simulink model "TemperatureControl"  (R2024b)
settings: Solver=FixedStepAuto  StartTime=0.0  StopTime=inf  FixedStep=0.1  RelTol=1e-3  EnableMultiTasking=on
libraries: arduinolib x6
settings Model: ExtModeTrigDuration=2  Creator=arkad  LastModifiedBy=arkad
settings SolverCC: AutoInsertRateTranBlk=on
settings OptimizationCC: EnhancedBackFolding=on  PassReuseOutputArgsAs=Individual arguments  ZeroExternalMemoryAtStartup=off  ZeroInternalMemoryAtStartup=off  MaxStackSize=64  OptimizeBlockOrder=speed  DifferentSizesBufferReuse=on  OptimizationCustomize=off  EfficientTunableParamExpr=on
settings DebuggingCC: ParameterTunabilityLossMsg=error
settings HardwareCC: ProdBitPerInt=16  ProdBitPerPointer=16  ProdBitPerSizeT=16  ProdBitPerPtrDiffT=16  ProdLargestAtomicFloat=None  ProdWordSize=8  ProdHWDeviceType=Atmel->AVR
settings SFSimCC: MATLABDynamicMemAlloc=off
settings RTWCC: Description=Embedded Coder  SystemTargetFile=ert.tlc  HardwareBoard=Arduino Uno  TemplateMakefile=ert_default_tmf  Toolchain=Arduino AVR  BuildConfiguration=Faster Runs
settings CodeAppCC: ForceParamTrailComments=on  IgnoreCustomStorageClasses=off  OperatorAnnotations=on  SimulinkDataObjDesc=on  SFDataObjDesc=on  InsertBlockDesc=on
settings ERTTargetCC: SupportContinuousTime=on  SupportVariableSizeSignals=on  ExtModeTransport=3  ExtModeStaticAlloc=on  ExtModeAutomaticAllocSize=off  ExtModeStaticAllocSize=250  ExtModeMexFile=ext_xcp  ExtModeIntrfLevel=Level2 - Open  InlinedParameterPlacement=Hierarchical

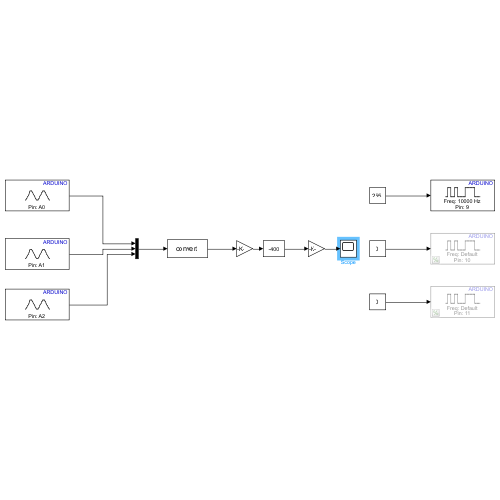
[thumbnail: Simulink's stored preview of the top-level diagram]
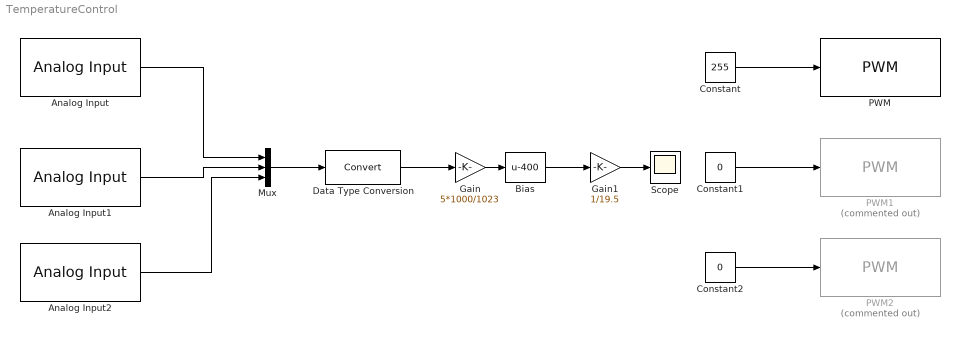
== system TemperatureControl ==
  Analog Input : arduinolib/Analog Input  pinNumber=0  ReadResultsOnly=off  ConversionTriggerSource=Software  ExternalTriggerType=uint32( 0 )  OutputDataType=uint16  EnableConversionCompleteNotify=off  EnableOuputStatus=off  SampleTime=-1  blockPlatform=arduino
      settings: SourceProductName=Common
  Analog Input1 : arduinolib/Analog Input  pinNumber=1  ReadResultsOnly=off  ConversionTriggerSource=Software  ExternalTriggerType=uint32( 0 )  OutputDataType=uint16  EnableConversionCompleteNotify=off  EnableOuputStatus=off  SampleTime=-1  blockPlatform=arduino
      settings: SourceProductName=Common
  Analog Input2 : arduinolib/Analog Input  pinNumber=2  ReadResultsOnly=off  ConversionTriggerSource=Software  ExternalTriggerType=uint32( 0 )  OutputDataType=uint16  EnableConversionCompleteNotify=off  EnableOuputStatus=off  SampleTime=-1  blockPlatform=arduino
      settings: SourceProductName=Common
  Bias : Bias  Bias=-400  SaturateOnIntegerOverflow=off
  Constant : Constant  Value=255
  Constant1 : Constant  Value=0
  Constant2 : Constant  Value=0
  Data Type Conversion : DataTypeConversion  SaturateOnIntegerOverflow=off  RndMeth=Floor
  Gain : Gain  Gain=5*1000/1023
  Gain1 : Gain  Gain=1/19.5
  Mux : Mux  Inputs=3
  PWM : arduinolib/PWM  pinNumber=9  frequencyType=Specify  desiredFrequency=10000  achievableFrequency=10000
      settings: SourceProductName=Common
  PWM1 : arduinolib/PWM  Commented=on  pinNumber=10  frequencyType=Default  desiredFrequency=490.2  achievableFrequency=490.2
      settings: SourceProductName=Common
  PWM2 : arduinolib/PWM  Commented=on  pinNumber=11  frequencyType=Default  desiredFrequency=490.2  achievableFrequency=490.2
      settings: SourceProductName=Common
  Scope : Scope
  wires:
  Constant2/1 -> PWM2/1
  Constant1/1 -> PWM1/1
  Constant/1 -> PWM/1
  Analog Input1/1 -> Mux/2
  Analog Input2/1 -> Mux/3
  Analog Input/1 -> Mux/1
  Mux/1 -> Data Type Conversion/1
  Gain1/1 -> Scope/1
  Gain/1 -> Bias/1
  Bias/1 -> Gain1/1
  Data Type Conversion/1 -> Gain/1
